simulink model "SITRA_Deadtime_Testbench"  (R2026a)
settings: Solver=FixedStepDiscrete  StopTime=0.0006  FixedStep=1e-06
settings Model: Creator=saisi  LastModifiedBy=saisi

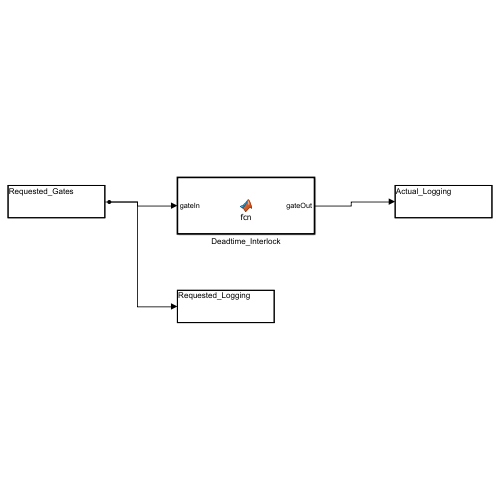
[thumbnail: Simulink's stored preview of the top-level diagram]
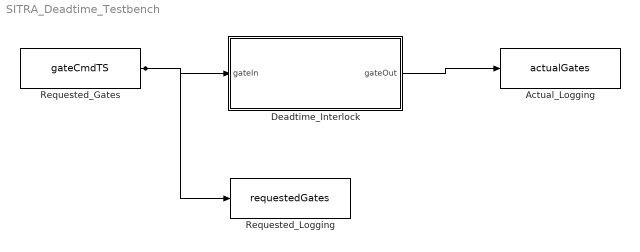
== system SITRA_Deadtime_Testbench ==
  Actual_Logging : ToWorkspace  VariableName=actualGates  SaveFormat=Timeseries  SampleTime=-1
  Deadtime_Interlock : MATLAB Function  TreatAsAtomicUnit=on
  Requested_Gates : FromWorkspace  VariableName=gateCmdTS  Interpolate=off  OutputAfterFinalValue=Holding final value
  Requested_Logging : ToWorkspace  VariableName=requestedGates  SaveFormat=Timeseries  SampleTime=-1
  wires:
  Requested_Gates/1 -> Deadtime_Interlock/1(gateIn), Requested_Logging/1
  Deadtime_Interlock/1(gateOut) -> Actual_Logging/1

== matlab function SITRA_Deadtime_Testbench/Deadtime_Interlock ==
  data: gateIn input; gateOut output
function gateOut = fcn(gateIn)

% Three-channel break-before-make interlock
% Ts = 1 us; dead-time = 5 us

persistent lastDesired blankCount initialized

if isempty(initialized)
    lastDesired = double(0);
    blankCount = double(0);
    initialized = true;
end

gateOut = zeros(1,3);

g1 = gateIn(1);
g2 = gateIn(2);
g3 = gateIn(3);

binaryValid = (g1==0 || g1==1) && (g2==0 || g2==1) && (g3==0 || g3==1);
exclusiveValid = (g1 + g2 + g3) <= 1;

if ~(binaryValid && exclusiveValid)
    blankCount = double(5);
    lastDesired = double(0);
    return;
end

desired = double(0);
if g1 == 1
    desired = double(1);
elseif g2 == 1
    desired = double(2);
elseif g3 == 1
    desired = double(3);
end

if desired ~= lastDesired
    blankCount = double(5);
    lastDesired = desired;
end

if blankCount > 0
    blankCount = blankCount - 1;
    return;
end

if desired == 1
    gateOut(1) = 1;
elseif desired == 2
    gateOut(2) = 1;
elseif desired == 3
    gateOut(3) = 1;
end

end
